simulink model "Braccio_CtrlSimMdl_2025b"  (R2025b)
settings: Solver=ode1  StartTime=0.0  StopTime=inf  FixedStep=dt  RelTol=1e-3  EnableMultiTasking=on
values from neighbouring files (symbols this model uses):
  dt = 0.01    [Braccio_ini.m]    (also in Braccio_kinematics.m)
  jnt1 = rigidBodyJoint('jnt1','revolute')    [Braccio_ini.m]    (also in Braccio_kinematics.m)
  jnt2 = rigidBodyJoint('jnt2','revolute')    [Braccio_ini.m]    (also in Braccio_kinematics.m)
  jnt3 = rigidBodyJoint('jnt3','revolute')    [Braccio_ini.m]    (also in Braccio_kinematics.m)
  jnt4 = rigidBodyJoint('jnt4','revolute')    [Braccio_ini.m]    (also in Braccio_kinematics.m)
  jnt5 = rigidBodyJoint('jnt5','revolute')    [Braccio_ini.m]    (also in Braccio_kinematics.m)
undefined symbols (not defined in the file or in its folder): DiscIntNeverNeededParam, efence1_coord, Gripper, Pause, Run
libraries: sim3dlib x22, Braccio_lib x12, simulink x12, robotmaniplib x1, stm32f4xxblockslib x1, robotcorelib x1, robotsim3dlib x1
(part 1 of 2)
settings Model: STM32="{\"DigitalPortRead\":[{\"ID\":\"MotorCtrl_Demo_STM32:8\"},{\"ID\":\"DemoSetup_H755ZIQ:8\"},{\"ID\":\"DemoSetup_H755ZIQ_M7:8\"},{\"ID\":\"Aktorik_H755ZIQ_M7:8\"},{\"ID\":\"IKS4A1_H755ZIQ_M7:8\"},{\"ID\":\"BlinkModel:8\"}],\"DigitalPortWrite\":[{\"ID\":\"MotorCtrl_Demo_STM32:9\"},{\"ID\":\"MotorCtrl_Demo_STM32:26\"},{\"ID\":\"MotorCtrl_Demo_STM32:27\"},{\"ID\":\"MotorCtrl_Demo_STM32:39\"},{\"ID\":\"MotorCtrl_Demo_STM32:489\"},{\"ID\":\"MotorCtrl_Demo_STM32:493\"},{\"ID\":\"MotorCtrl_Demo_STM32:582\"},{\"ID\":\"MotorCtrl_Demo_STM32:584\"},{\"ID\":\"MotorCtrl_Demo_STM32:585\"},{\"ID\":\"MotorCtrl_Demo_STM32:586\"},{\"ID\":\"DemoSetup_H755ZIQ:9\"},{\"ID\":\"DemoSetup_H755ZIQ_M7:9\"},{\"ID\":\"Aktorik_H755ZIQ_M7:9\"},{\"ID\":\"Aktorik_H755ZIQ_M7:886\"},{\"ID\":\"Aktorik_H755ZIQ_M7:887\"},{\"ID\":\"Aktorik_H755ZIQ_M7:929\"},{\"ID\":\"Aktorik_H755ZIQ_M7:930\"},{\"ID\":\"Aktorik_H755ZIQ_M7:1123\"},{\"ID\":\"Aktorik_H755ZIQ_M7:1128\"},{\"ID\":\"Aktorik_H755ZIQ_M7:1152\"},{\"ID\":\"Aktorik_H755ZIQ_M7:1176\"},{\"ID\":\"Aktorik_H755ZIQ_M7:1222\"},{\"ID\":\"Aktorik_H755ZIQ_M7:1224\"},{\"ID\":\"Aktorik_H755ZIQ_M7:1233\"},{\"ID\":\"IKS4A1_H755ZIQ_M7:9\"},{\"ID\":\"BlinkModel:9\"},{\"ID\":\"2666\"},{\"ID\":\"Braccio_CtrlSimMdl_2025b:2666\"}],\"PWMOutput\":[{\"ID\":\"MotorCtrl_Demo_STM32:23\"},{\"ID\":\"Aktorik_H755ZIQ_M7:885\"},{\"ID\":\"Aktorik_H755ZIQ_M7:988\"}],\"EncoderBlock\":[{\"ID\":\"MotorCtrl_Demo_STM32:41\"},{\"ID\":\"Aktorik_H755ZIQ_M7:1005\"}],\"AnalogInputForH7\":{\"ID\":\"Aktorik_H755ZIQ_M7:875\"},\"I2CControllerRead\":[{\"ID\":\"Aktorik_H755ZIQ_M7:1322\"},{\"ID\":\"Aktorik_H755ZIQ_M7:1414\"},{\"ID\":\"Aktorik_H755ZIQ_M7:1416\"},{\"ID\":\"Aktorik_H755ZIQ_M7:1435\"},{\"ID\":\"Aktorik_H755ZIQ_M7:1437\"},{\"ID\":\"Aktorik_H755ZIQ_M7:1438\"},{\"ID\":\"Aktorik_H755ZIQ_M7:1465\"},{\"ID\":\"Aktorik_H755ZIQ_M7:1466\"},{\"ID\":\"Aktorik_H755ZIQ_M7:1488\"},{\"ID\":\"Aktorik_H755ZIQ_M7:1489\"},{\"ID\":\"Aktorik_H755ZIQ_M7:1491\"},{\"ID\":\"Aktorik_H755ZIQ_M7:1492\"},{\"ID\":\"Aktorik_H755ZIQ_M7:1495\"},{\"ID\":\"Aktorik_H755ZIQ_M7:1496\"},{\"ID\":\"Aktorik_H755ZIQ_M7:1497\"},{\"ID\":\"Aktorik_H755ZIQ_M7:1498\"},{\"ID\":\"Aktorik_H755ZIQ_M7:1499\"},{\"ID\":\"Aktorik_H755ZIQ_M7:1500\"},{\"ID\":\"IKS4A1_H755ZIQ_M7:1435\"},{\"ID\":\"IKS4A1_H755ZIQ_M7:1437\"},{\"ID\":\"IKS4A1_H755ZIQ_M7:1438\"},{\"ID\":\"IKS4A1_H755ZIQ_M7:1414\"},{\"ID\":\"IKS4A1_H755ZIQ_M7:1416\"},{\"ID\":\"IKS4A1_H755ZIQ_M7:1495\"},{\"ID\":\"IKS4A1_H755ZIQ_M7:1496\"},{\"ID\":\"IKS4A1_H755ZIQ_M7:1497\"},{\"ID\":\"IKS4A1_H755ZIQ_M7:1498\"},{\"ID\":\"IKS4A1_H755ZIQ_M7:1499\"},{\"ID\":\"IKS4A1_H755ZIQ_M7:1500\"},{\"ID\":\"IKS4A1_H755ZIQ_M7:1465\"},{\"ID\":\"IKS4A1_H755ZIQ_M7:1466\"},{\"ID\":\"IKS4A1_H755ZIQ_M7:1488\"},{\"ID\":\"IKS4A1_H755ZIQ_M7:1489\"},{\"ID\":\"IKS4A1_H755ZIQ_M7:1491\"},{\"ID\":\"IKS4A1_H755ZIQ_M7:1492\"}],\"I2CControllerWrite\":[{\"ID\":\"Aktorik_H755ZIQ_M7:1375\"},{\"ID\":\"Aktorik_H755ZIQ_M7:1404\"},{\"ID\":\"Aktorik_H755ZIQ_M7:1452\"},{\"ID\":\"Aktorik_H755ZIQ_M7:1459\"},{\"ID\":\"Aktorik_H755ZIQ_M7:1511\"},{\"ID\":\"IKS4A1_H755ZIQ_M7:1404\"},{\"ID\":\"IKS4A1_H755ZIQ_M7:1375\"},{\"ID\":\"IKS4A1_H755ZIQ_M7:1452\"},{\"ID\":\"IKS4A1_H755ZIQ_M7:1511\"},{\"ID\":\"IKS4A1_H755ZIQ_M7:1459\"}]}"  ExtModeTrigDuration=10  Creator=bende  LastModifiedBy=natte
settings SolverCC: AutoInsertRateTranBlk=on
settings OptimizationCC: EnhancedBackFolding=on  PassReuseOutputArgsThreshold=0.0  MaxStackSize=256  OptimizeBlockOrder=speed  DifferentSizesBufferReuse=on  OptimizationCustomize=off
settings DebuggingCC: ParameterTunabilityLossMsg=error
settings HardwareCC: ProdBitPerLong=64.0  ProdHWDeviceType=Intel->x86-64 (Linux 64)  TargetBitPerPointer=64.0  TargetBitPerSizeT=64.0  TargetBitPerPtrDiffT=64.0  TargetLongLongMode=on  TargetIntDivRoundTo=Zero  TargetEndianess=LittleEndian  TargetWordSize=64.0  TargetHWDeviceType=MATLAB Host  ProdEqTarget=off
settings SFSimCC: MATLABDynamicMemAlloc=off
settings RTWCC: SystemTargetFile=rsim.tlc  TemplateMakefile=rsim_default_tmf  Toolchain=GNU Tools for ARM Embedded Processors  Description=Rapid Simulation Target
settings CodeAppCC: ForceParamTrailComments=on  MaxIdLength=95.0  OperatorAnnotations=on
settings STFCustomTargetCC: SystemTargetFile=rsim.tlc  TargetLangStandard=C99 (ISO)  ModelReferenceCompliant=off  ConcurrentExecutionCompliant=off  MATLABClassNameForMDSCustomization=Simulink.SoftwareTarget.TargetSpecificTriggerConfigurationBase
settings RSimTargetCC: ExtModeStaticAllocSize=1000000.0  ExtModeTransport=0.0  MultiwordLength=2048.0

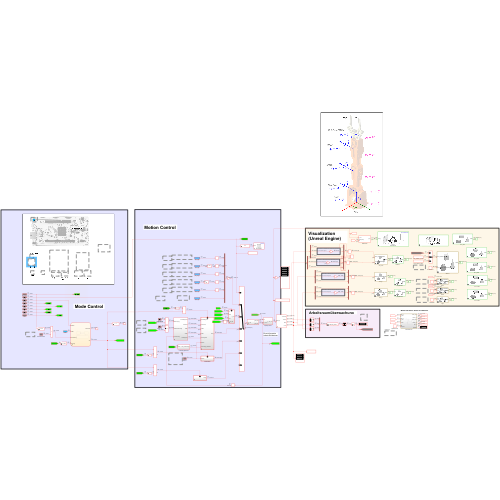
[thumbnail: Simulink's stored preview of the top-level diagram]
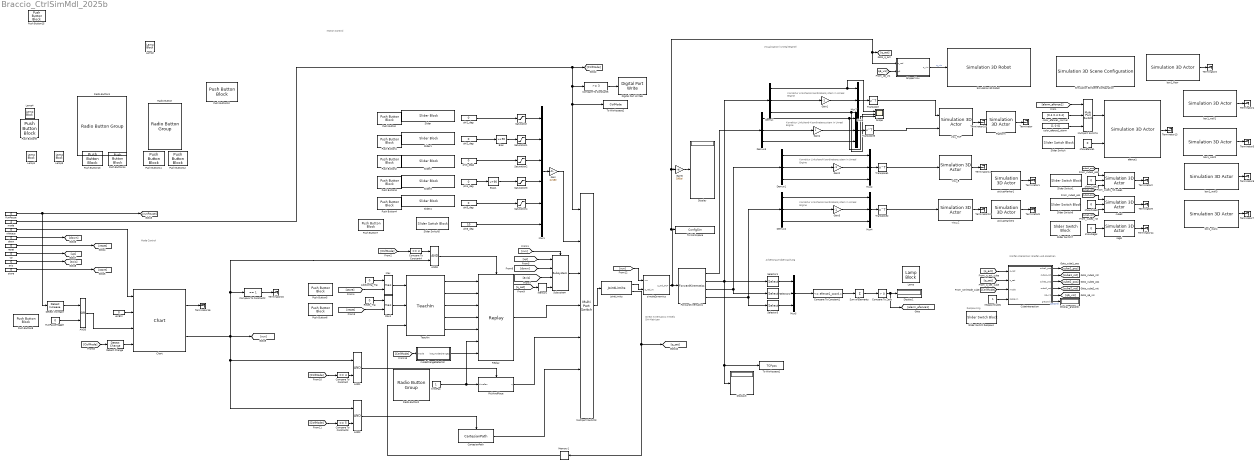
== system Braccio_CtrlSimMdl_2025b ==
  note: Korrektur Linkshand-Koordinatensystem
      | in Unreal Engine
  note: Arbeitsraumüberwachung
  note: Korrektur Linkshand-Koordinatensystem
      | in Unreal Engine
  note: Korrektur Linkshand-Koordinatensystem
      | in Unreal Engine
  note: Visualization
      | (Unreal Engine)
  note: Korrektur Linkshand-Koordinatensystem
      | in Unreal Engine
  note: Mode Control
  note: Motion Control
  note: Direct Kinematics
      | mittels DH-Matrizen
  note: Würfel-Interaktion: Greifen und Absetzen
  note: Respawning
  AND1 : Logic  AllPortsSameDT=off  OutDataTypeStr=boolean
  AND2 : Logic  AllPortsSameDT=off  OutDataTypeStr=boolean
  AND3 : Logic  AllPortsSameDT=off  OutDataTypeStr=boolean
  AND5 : Logic  Operator=OR  AllPortsSameDT=off  OutDataTypeStr=boolean
  AddConfig_Trg : Constant  Value=0  SampleTime=dt
  Bias : Bias  Bias=90  SaturateOnIntegerOverflow=off
  Bias1 : Bias  Bias=90  SaturateOnIntegerOverflow=off
  CartesianPath : Braccio_lib/CartesianPath  SystemSampleTime=-1  VariantActivationTime=update diagram  EmptyChoice=off  PassThrough=off  PassThroughVariantControl=(default)  EmptyChoiceVariantControl=(default)  AllowFlexibleInterface=on  Latency=0  AutoFrameSizeCalculation=off
  Chart : Braccio_lib/Chart  SystemSampleTime=-1  VariantActivationTime=update diagram  EmptyChoice=off  PassThrough=off  PassThroughVariantControl=(default)  EmptyChoiceVariantControl=(default)  AllowFlexibleInterface=on  Latency=0  AutoFrameSizeCalculation=off
  Compare To Constant : simulink/Logic and Bit Operations/Compare To Constant  relop===  const=4  OutDataTypeStr=boolean
  Compare To Constant1 : simulink/Logic and Bit Operations/Compare To Constant  relop=<=  const=efence1_coord.x  OutDataTypeStr=boolean
  Compare To Constant2 : simulink/Logic and Bit Operations/Compare To Constant  relop===  const=1  OutDataTypeStr=boolean
  Compare To Constant3 : simulink/Logic and Bit Operations/Compare To Constant  relop===  const=5  OutDataTypeStr=boolean
  Compare To Constant4 : simulink/Logic and Bit Operations/Compare To Constant  relop===  const=3  OutDataTypeStr=boolean
  Compare To Constant5 : simulink/Logic and Bit Operations/Compare To Constant  relop=>=  const=3  OutDataTypeStr=boolean
  Compare To Zero : simulink/Logic and Bit Operations/Compare To Zero  relop=>  OutDataTypeStr=boolean
  CubeInteraction : Subsystem
  Demux{,1..3} (4 alike) : Demux  Outputs=3
  Detect Change : simulink/Logic and Bit Operations/Detect Change  vinit=0  OutDataTypeStr=boolean
  Detect Increase : simulink/Logic and Bit Operations/Detect Increase  vinit=0.0  OutDataTypeStr=boolean
  Digital Port Write5 : stm32f4xxblockslib/Digital Port Write  PortName=GPIOD  PinNumber=7  ReadOperation=off  IOAsArray=off  EnableSimPort=off  hoistedMaskSrc=ECSoC/ECSimCodegen/Digital Port Write
      settings: LibrarySourceBlock=stm32h7xxblockslib/Digital Port Write
  Display : Display
  Display1 : Display
  Display3 : Display
  Display_graspIdx : Display
  ForwardKinematics : Braccio_lib/ForwardKinematics  SystemSampleTime=-1  VariantActivationTime=update diagram  EmptyChoice=off  PassThrough=off  PassThroughVariantControl=(default)  EmptyChoiceVariantControl=(default)  AllowFlexibleInterface=on  Latency=0  AutoFrameSizeCalculation=off
  Gain : Gain  Gain=pi/180
  Gain1 : Gain  Gain=-1
  Gain2 : Gain  Gain=-1
  Gain3 : Gain  Gain=-1
  Gain4 : Gain
  Gain5 : Gain  Gain=180/pi
  GripperVisu : MATLAB Function  TreatAsAtomicUnit=on
  JointLimits : Braccio_lib/JointLimits  SystemSampleTime=-1  VariantActivationTime=update diagram  EmptyChoice=off  PassThrough=off  PassThroughVariantControl=(default)  EmptyChoiceVariantControl=(default)  AllowFlexibleInterface=on  Latency=0  AutoFrameSizeCalculation=off
  Lamp{,1..4} (5 alike) : LampBlock  LabelPosition=Hide  DefaultColor=[192.0, 192.0, 192.0]
  Max : MinMax  Function=max  Inputs=2
  Max1 : MinMax  Function=max  Inputs=2
  Memory : Memory  InitialCondition=[0;90;0;90;0;20]*pi/180
  Memory1 : Memory  InheritSampleTime=on
  Multiport Switch1 : MultiPortSwitch  DataPortOrder=Zero-based contiguous  Inputs=2  zeroidx=on  SaturateOnIntegerOverflow=off  InputSameDT=off
  Multiport Switch3 : MultiPortSwitch  Inputs=6  SaturateOnIntegerOverflow=off  InputSameDT=off
  Mux1 : Mux  Inputs=6
  Mux{2..5,7} (5 alike) : Mux  Inputs=3
  PickAndPlace : Subsystem  AncestorBlock=Braccio_lib/PickAndPlace
  Platform : sim3dlib/Simulation 3D Actor  Priority=1  ActorName=actor1_platform  ParentName=Scene Origin  Operation=Create at setup  InitScriptText=|  SampleTime=-1  Translation=[0.1 0 -0.01]  Rotation=[0 0 0]  Scale=[1 1 1]  aMode=5  ActorTag=actor1_platform  ActorType=Sim3dActor  ID=C
      | % Reserved keywords:
      | % - Actor : handle to this actor object
      | % - World : handle to the world object
      | 
      | % Examples:
      | 
      | % Create a primitive geometry (optional)
      | createShape(Actor, 'box', [0.6,0.3,0.02]);
      | 
      | % Initialize values (optional)
      | Actor.Physics = false;
      | Actor.Color = [0.4 0.4 0.4];
      | %platform = collisionBox(0.6,0.3,0.02);
      | %platform.Pose = trvec2tform([-0.1 0 -.01]);
  Push Button : PushButtonBlock  ButtonText=Reset q1  OnValue=0  ButtonType=Latch  IconOnColor=[0.0, 0.39215686274509803, 0.0]  IconOffColor=[0.0, 1.0, 0.0]  OffValue=-2.550607
  Push Button1 : PushButtonBlock  ButtonText=Reset q2  OnValue=0  ButtonType=Latch  IconOnColor=[0.0, 0.39215686274509803, 0.0]  IconOffColor=[0.0, 1.0, 0.0]  OffValue=48.947368
  Push Button10 : PushButtonBlock  ButtonText=NOTAUS  Icon=Circle  IconOnColor=[1.0, 0.0, 0.0]  IconOffColor=[1.0, 0.0, 0.0]  IconColor=On  OffValue=0.000000
  Push Button{9,11..14} (5 alike) : PushButtonBlock  Icon=Circle  IconOnColor=[0.0, 0.39215686274509803, 0.0]  IconOffColor=[0.0, 1.0, 0.0]  OffValue=0.000000
  Push Button15 : PushButtonBlock  ButtonText=USR BTN  IconOnColor=[0.0, 0.39215686274509803, 0.0]  IconOffColor=[0.0, 1.0, 0.0]  OffValue=0.000000
  Push Button2 : PushButtonBlock  ButtonText=Reset q3  OnValue=0  ButtonType=Latch  IconOnColor=[0.0, 0.39215686274509803, 0.0]  IconOffColor=[0.0, 1.0, 0.0]  OffValue=-17.636995
  Push Button3 : PushButtonBlock  ButtonText=Reset q4  OnValue=0  ButtonType=Latch  IconOnColor=[0.0, 0.39215686274509803, 0.0]  IconOffColor=[0.0, 1.0, 0.0]  OffValue=-12.105263
  Push Button4 : PushButtonBlock  ButtonText=Reset q5  OnValue=0  ButtonType=Latch  IconOnColor=[0.0, 0.39215686274509803, 0.0]  IconOffColor=[0.0, 1.0, 0.0]  OffValue=-61.435656
  Push Button5 : PushButtonBlock  ButtonText=SAVE CONFIG  IconOnColor=[0.0, 0.39215686274509803, 0.0]  IconOffColor=[0.0, 1.0, 0.0]  OffValue=0.000000
  Push Button6 : PushButtonBlock  ButtonText=RESET  IconOnColor=[0.0, 0.39215686274509803, 0.0]  IconOffColor=[0.0, 1.0, 0.0]
  Push Button7 : PushButtonBlock  ButtonText=SAVE CONFIG  IconOnColor=[0.0, 0.39215686274509803, 0.0]  IconOffColor=[0.0, 1.0, 0.0]  OffValue=0.000000
  Push Button8 : PushButtonBlock  ButtonText=Run-Pause  IconOnColor=[0.0, 0.39215686274509803, 0.0]  IconOffColor=[0.0, 1.0, 0.0]  OffValue=0.000000
  Radio Button : RadioButtonGroup  LabelPosition=Hide  SelectedLabel=6 - Gripper  ButtonGroupName=Axis
  Radio Button1 : RadioButtonGroup  LabelPosition=Hide  SelectedLabel=Pick'n'Place  ButtonGroupName=Mode
  Radio Button2 : RadioButtonGroup  LabelPosition=Hide  SelectedLabel=Normal  ButtonGroupName=timeFac
  Replay : Braccio_lib/Replay  SystemSampleTime=-1  VariantActivationTime=update diagram  EmptyChoice=off  PassThrough=off  PassThroughVariantControl=(default)  EmptyChoiceVariantControl=(default)  AllowFlexibleInterface=on  Latency=0  AutoFrameSizeCalculation=off
  Reset_Trg : Constant  Value=0  SampleTime=dt
  RunPause : Constant  Value=0  SampleTime=dt
  RunPauseToggle : Constant  Value=0  SampleTime=dt
  Saturation : Saturate  UpperLimit=jnt1.PositionLimits(2)*180/pi  LowerLimit=jnt1.PositionLimits(1)*180/pi
  Saturation1 : Saturate  UpperLimit=jnt2.PositionLimits(2)*180/pi  LowerLimit=jnt2.PositionLimits(1)*180/pi
  Saturation2 : Saturate  UpperLimit=jnt3.PositionLimits(2)*180/pi  LowerLimit=jnt3.PositionLimits(1)*180/pi
  Saturation3 : Saturate  UpperLimit=jnt4.PositionLimits(2)*180/pi  LowerLimit=jnt4.PositionLimits(1)*180/pi
  Saturation4 : Saturate  UpperLimit=jnt5.PositionLimits(2)*180/pi  LowerLimit=jnt5.PositionLimits(1)*180/pi
  Scope : Scope  NumInputPorts=3
      settings: ActiveDisplayYMinimum=0.35929394467848708  ActiveDisplayYMaximum=0.36634551278284788  DataLoggingVariableName=ScopeData3
  Selector1 : Selector  InputPortWidth=3  IndexOptions=Index vector (dialog)  Indices=1  OutputSizes=1
  Selector2 : Selector  InputPortWidth=3  IndexOptions=Index vector (dialog)  Indices=1  OutputSizes=1
  Selector3 : Selector  InputPortWidth=3  IndexOptions=Index vector (dialog)  Indices=1  OutputSizes=1
  Simulation 3D Robot : robotsim3dlib/Simulation 3D Robot  actorInputType=RigidBodyTree Object  RigidBodyTree=braccioRobotVis  ActorName=braccioRobot  existActorChekBox=off  initialTrans=[0 0 0]  initialRot=[0 0 0]  initialConfig=braccioInitConfigVis  EndEffector=body5  eeOffsetInpChekBox=off  eeTargetTrans=[0 0 0]  eeTargetRot=[0 0 0]  enableRegionGraspChekBox=off  regionGraspInpChekBox=off  eeTargTransDiff=[0.2 0.2 0.2]  eeTargRotDiff=[0 0 0]  enableVisualVisualization=on  enableCollisionVisualization=on  collisionGeomColor=[0 1 0]  collisionGeomTransp=0.1  inpConfEnbVal=on  inpGraspEnbVal=off  inpTransEnbVal=off  outConfEnbVal=off  outGraspEnbVal=off  outTransEnbVal=off  SampleTime=-1  ActorType=SimulinkVehicle  ID=C  aMode=6  ActorTag=braccioRobot  Mesh=RigidBodyTree
  Simulation 3D Scene Configuration : sim3dlib/Simulation 3D Scene Configuration  Priority=0  ProjectFormat=Default Scenes  SceneDesc=Empty scene  ProjectName=C:\Program Files\MATLAB\R2025b\toolbox\shared\sim3d_projects\automotive_project_windows\UE\WindowsNoEditor\VehicleSimulation.exe  ScenePath=/Game/Maps/EmptyScene  EnableOpenDRIVE=off  vehTagList={'Actor_B';'Actor_C';'Actor_TCP';'Actor_efence1';'Custom';'Scene Origin';'Sim3dActor1';'View1';'View2';'View3';'View4';'actor1_platform';'actor2_pickupMarker';'actor_cube1';'actor_cube2';'actor_regal';'boxActor1';'boxActor2';'boxActor3';'boxActor4';'boxActor5';'braccioRobot'}  vehTag=View4  AttachedCameraRelativeTranslation=[0 0 0]  FreeCameraDefaultInitialTranslation=[-6, 0, 2]  AttachedCameraRelativeRotation=[0 0 0]  FreeCameraDefaultInitialRotation=[0, -15, 0]  ViewpointName=View4  FreeCameraInitialTranslation=[0.25 -0.4 0.4]  ViewpointTranslation=[0 0 0]  FreeCameraInitialRotation=[0 -35 110]  ViewpointRotation=[0 0 0]  OpVisEn=off  Ts=0.1  EnableWindow=on  EnableRemoteAccess=off  EnableWeather=on  SunAzimuth=90  SunAltitude=40.0  EnableGeospatialSun=off  Latitude=0  Longitude=0  Date=2023-01-01  Time=10:30:00  GeoTimeZone=-5.0  SunDaylightSaving=off  wind=0  clouds=0.0  EnableVolumetricClouds=off  CloudCoverage=0  CloudAltitude=6  fog=0  rain=0  RaindropsEffect=off  SnowDensity=0  EnableGeospatial=off  TilesetSource=Earth terrain  UseTrueOrigin=off  OriginHeight=200  OriginLatitude=40.744652  OriginLongitude=-73.988864  MapStyle=Aerial  AdditionalAssetIDs=[]  UseAdvancedSunSky=off  SolarTime=11  TimeZone=-5  Day=21  Month=9  Year=2022  UseDaylightSavingTime=on  DSTStartDay=10  DSTStartMonth=3  DSTEndDay=3  DSTEndMonth=11  DSTSwitchHour=2  sensorTag=MainCamera1  sensorId=1  sensorName=MainCamera1  mountLoc=Origin  offsetFlag=off  tmountOffset=[0, 0, 0]  rmountOffset=[0, 0, 0]  HorizontalResolution=1280  VerticalResolution=720  HorizontalFOV=60  mountPoint=[0 0 0]  mountOrientation=[0 0 0]  aMode=6  ID=1  GeoTrigger=Inactive  ViewNameList={'Custom', 'View1', 'View2', 'View3', 'View4'}  ViewTranslationList={'[0 -1 0]', '[-0.5 0 0.05]', '[0 -0.5 0.05]', '[0.15 0.5 0.25]', '[0.25 -0.4 0.4]'}  ViewRotationList={'[0 0 0]', '[0 0 0]', '[0 0 90]', '[0 -5 -90]', '[0 -35 110]'}
      settings: LibrarySourceBlock=robotsim3dlib/Simulation 3D Scene Configuration
  Slider{,1..4} (5 alike) : SliderBlock  ScaleMin=-90  ScaleMax=90
  Slider Switch{,1,5..7} (5 alike) : SliderSwitchBlock
  Slider Switch Respawn : SliderSwitchBlock
  Subsystem : Braccio_lib/Subsystem  SystemSampleTime=-1  VariantActivationTime=update diagram  EmptyChoice=off  PassThrough=off  PassThroughVariantControl=(default)  EmptyChoiceVariantControl=(default)  AllowFlexibleInterface=on  Latency=0  AutoFrameSizeCalculation=off
  Sum of Elements : Sum  Inputs=+
  TeachIn : Braccio_lib/TeachIn  SystemSampleTime=-1  VariantActivationTime=update diagram  EmptyChoice=off  PassThrough=off  PassThroughVariantControl=(default)  EmptyChoiceVariantControl=(default)  AllowFlexibleInterface=on  Latency=0  AutoFrameSizeCalculation=off
  Terminator{,1..16} (17 alike) : Terminator
  To Workspace : ToWorkspace  VariableName=ConfigSim  SaveFormat=Timeseries  SampleTime=-1
  To Workspace1 : ToWorkspace  VariableName=TCPpos  SaveFormat=Timeseries  SampleTime=-1
  To Workspace2 : ToWorkspace  VariableName=CtrlMode  SaveFormat=Timeseries  SampleTime=-1
  Transpose{,1..3} (4 alike) : Math  Operator=transpose
  axis : Constant  Value=6  SampleTime=dt
  box1_floor : sim3dlib/Simulation 3D Actor  Priority=1  ActorName=boxActor2  ParentName=Scene Origin  Operation=Create at setup  InitScriptText=|  SampleTime=-1  Translation=[0 -0.225 -.015]  Rotation=[0 0 0]  Scale=[1 1 1]  aMode=5  ActorTag=boxActor2  ActorType=Sim3dActor  ID=C
      | % Reserved keywords:
      | % - Actor : handle to this actor object
      | % - World : handle to the world object
      | 
      | % Examples:
      | 
      | % Create a primitive geometry (optional)
      | createShape(Actor, 'box', [0.1,0.15,0.005]);
      | 
      | % Initialize values (optional)
      | Actor.Physics = false;
      | Actor.Color = [0.4 0.4 0.4];
      | %platform = collisionBox(0.6,0.3,0.02);
      | %platform.Pose = trvec2tform([-0.1 0 -.01]);
  box1_wall1 : sim3dlib/Simulation 3D Actor  Priority=1  ActorName=boxActor3  ParentName=Scene Origin  Operation=Create at setup  InitScriptText=|  SampleTime=-1  Translation=[0 -0.15 .05-0.02]  Rotation=[0 0 0]  Scale=[1 1 1]  aMode=5  ActorTag=boxActor3  ActorType=Sim3dActor  ID=C
      | % Reserved keywords:
      | % - Actor : handle to this actor object
      | % - World : handle to the world object
      | 
      | % Examples:
      | 
      | % Create a primitive geometry (optional)
      | createShape(Actor, 'box', [0.1,0.005,0.1]);
      | 
      | % Initialize values (optional)
      | Actor.Physics = false;
      | Actor.Color = [0.4 0.4 0.4];
      | %platform = collisionBox(0.6,0.3,0.02);
      | %platform.Pose = trvec2tform([-0.1 0 -.01]);
  box1_wall2 : sim3dlib/Simulation 3D Actor  Priority=1  ActorName=boxActor4  ParentName=Scene Origin  Operation=Create at setup  InitScriptText=|  SampleTime=-1  Translation=[0 -0.3 .05-0.02]  Rotation=[0 0 0]  Scale=[1 1 1]  aMode=5  ActorTag=boxActor4  ActorType=Sim3dActor  ID=C
      | % Reserved keywords:
      | % - Actor : handle to this actor object
      | % - World : handle to the world object
      | 
      | % Examples:
      | 
      | % Create a primitive geometry (optional)
      | createShape(Actor, 'box', [0.1,0.005,0.1]);
      | 
      | % Initialize values (optional)
      | Actor.Physics = false;
      | Actor.Color = [0.4 0.4 0.4];
      | %platform = collisionBox(0.6,0.3,0.02);
      | %platform.Pose = trvec2tform([-0.1 0 -.01]);
  box1_wall3 : sim3dlib/Simulation 3D Actor  Priority=1  ActorName=boxActor5  ParentName=Scene Origin  Operation=Create at setup  InitScriptText=|  SampleTime=-1  Translation=[0.05 -0.225 0.05-0.02]  Rotation=[0 0 0]  Scale=[1 1 1]  aMode=5  ActorTag=boxActor5  ActorType=Sim3dActor  ID=C
      | % Reserved keywords:
      | % - Actor : handle to this actor object
      | % - World : handle to the world object
      | 
      | % Examples:
      | 
      | % Create a primitive geometry (optional)
      | createShape(Actor, 'box', [0.005,0.15,0.1]);
      | 
      | % Initialize values (optional)
      | Actor.Physics = false;
      | Actor.Color = [0.4 0.4 0.4];
      | %platform = collisionBox(0.6,0.3,0.02);
      | %platform.Pose = trvec2tform([-0.1 0 -.01]);
  box1_wall4 : sim3dlib/Simulation 3D Actor  Priority=1  ActorName=boxActor1  ParentName=Scene Origin  Operation=Create at setup  InitScriptText=|  SampleTime=-1  Translation=[-0.05 -0.225 0.05-0.02]  Rotation=[0 0 0]  Scale=[1 1 1]  aMode=5  ActorTag=boxActor1  ActorType=Sim3dActor  ID=C
      | % Reserved keywords:
      | % - Actor : handle to this actor object
      | % - World : handle to the world object
      | 
      | % Examples:
      | 
      | % Create a primitive geometry (optional)
      | createShape(Actor, 'box', [0.005,0.15,0.1]);
      | 
      | % Initialize values (optional)
      | Actor.Physics = false;
      | Actor.Color = [0.4 0.4 0.4];
      | %platform = collisionBox(0.6,0.3,0.02);
      | %platform.Pose = trvec2tform([-0.1 0 -.01]);
  color_efence1_alarm : Constant  Value=[1 0 0]  SampleTime=dt
  color_efence1_normal : Constant  Value=[0.4 0.4 0.4]  SampleTime=dt
  cube1 : sim3dlib/Simulation 3D Actor  Priority=1  ActorName=actor_cube1  ParentName=Scene Origin  Operation=Create at setup  InitScriptText=|  SampleTime=-1  Translation=[0.25 0 0.025/2+0.005]  Rotation=[0 0 0]  Scale=[1 1 1]  InputsText=|  aMode=5  ActorTag=actor_cube1  ActorType=Sim3dActor  ID=C
      InitScriptText=|
      | % Reserved keywords:
      | % - Actor : handle to this actor object
      | % - World : handle to the world object
      | 
      | % Examples:
      | 
      | % Create a primitive geometry (optional)
      | createShape(Actor, 'box', [0.025,0.025,0.025]);
      | 
      | % Initialize values (optional)
      | Actor.Physics = false;
      | Actor.Color = [0 0 1];
      | %platform = collisionBox(0.6,0.3,0.02);
      | %platform.Pose = trvec2tform([-0.1 0 -.01]);
      InputsText=|
      | actor_cube1.Translation
      | actor_cube1.Transparency
      | actor_cube1.Rotation
  cube2 : sim3dlib/Simulation 3D Actor  Priority=1  ActorName=actor_cube2  ParentName=Scene Origin  Operation=Create at setup  InitScriptText=|  SampleTime=-1  Translation=[0.35 0 0.025/2+0.005]  Rotation=[0 0 0]  Scale=[1 1 1]  InputsText=|  aMode=5  ActorTag=actor_cube2  ActorType=Sim3dActor  ID=C
      InitScriptText=|
      | % Reserved keywords:
      | % - Actor : handle to this actor object
      | % - World : handle to the world object
      | 
      | % Examples:
      | 
      | % Create a primitive geometry (optional)
      | createShape(Actor, 'box', [0.025,0.025,0.025]);
      | 
      | % Initialize values (optional)
      | Actor.Physics = false;
      | Actor.Color = [0 1 0];
      | %platform = collisionBox(0.6,0.3,0.02);
      | %platform.Pose = trvec2tform([-0.1 0 -.01]);
      InputsText=|
      | actor_cube2.Translation
      | actor_cube2.Transparency
      | actor_cube2.Rotation
  down : Constant  Value=0  SampleTime=dt
  efence1 : sim3dlib/Simulation 3D Actor  Priority=1  ActorName=Actor_efence1  ParentName=Scene Origin  Operation=Create at setup  InitScriptText=|  SampleTime=-1  Translation=[efence1_coord.x 0 0.15]  Rotation=[0 0 0]  Scale=[1 1 1]  InputsText="Actor_efence1.Color        Actor_efence1.Transparency"  aMode=5  ActorTag=Actor_efence1  ActorType=Sim3dActor  ID=C
      | % Reserved keywords:
      | % - Actor : handle to this actor object
      | % - World : handle to the world object
      | 
      | % Examples:
      | 
      | % Create a primitive geometry (optional)
      | createShape(Actor, 'box', [0.002,0.3,0.3]);
      | 
      | % Initialize values (optional)
      | Actor.Physics = false;
      | Actor.Color = [0.4 0.4 0.4];
      | Actor.Transparency = 0.4;
      | %platform = collisionBox(0.6,0.3,0.02);
      | %platform.Pose = trvec2tform([-0.1 0 -.01]);
  mode : Constant  Value=4  SampleTime=dt
  modeChangeDetector : Subsystem
  phi1_deg : Constant  Value=0  SampleTime=dt
  phi2_deg : Constant  Value=0  VectorParams1D=off  SampleTime=dt
  phi3_deg1 : Constant  Value=0  SampleTime=dt
  phi4_deg : Constant  Value=0  SampleTime=dt
  phi5_deg : Constant  Value=0  SampleTime=dt
  phi6_deg : Constant  Value=10  SampleTime=dt
  pickupMarker1 : sim3dlib/Simulation 3D Actor  Priority=1  ActorName=actor2_pickupMarker  ParentName=Scene Origin  Operation=Create at setup  InitScriptText=|  SampleTime=-1  Translation=[0.25 0 -.005]  Rotation=[0 0 0]  Scale=[1 1 1]  aMode=5  ActorTag=actor2_pickupMarker  ActorType=Sim3dActor  ID=C
      | % Reserved keywords:
      | % - Actor : handle to this actor object
      | % - World : handle to the world object
      | 
      | % Examples:
      | 
      | % Create a primitive geometry (optional)
      | createShape(Actor, 'box', [0.025,0.025,0.012]);
      | 
      | % Initialize values (optional)
      | Actor.Physics = false;
      | Actor.Color = [0.3 0.3 0.3];
      | %platform = collisionBox(0.6,0.3,0.02);
      | %platform.Pose = trvec2tform([-0.1 0 -.01]);
  pickupMarker2 : sim3dlib/Simulation 3D Actor  Priority=1  ActorName=Sim3dActor1  ParentName=Scene Origin  Operation=Create at setup  InitScriptText=|  SampleTime=-1  Translation=[0.35 0 -.005]  Rotation=[0 0 0]  Scale=[1 1 1]  aMode=5  ActorTag=Sim3dActor1  ActorType=Sim3dActor  ID=1
      | % Reserved keywords:
      | % - Actor : handle to this actor object
      | % - World : handle to the world object
      | 
      | % Examples:
      | 
      | % Create a primitive geometry (optional)
      | createShape(Actor, 'box', [0.025,0.025,0.012]);
      | 
      | % Initialize values (optional)
      | Actor.Physics = false;
      | Actor.Color = [0.3 0.3 0.3];
      | %platform = collisionBox(0.6,0.3,0.02);
      | %platform.Pose = trvec2tform([-0.1 0 -.01]);
  regal : sim3dlib/Simulation 3D Actor  Priority=1  ActorName=actor_regal  ParentName=Scene Origin  Operation=Create at setup  InitScriptText=|  SampleTime=-1  Translation=[0.4 0 0.05]  Rotation=[0 0 0]  Scale=[1 1 1]  InputsText=actor_regal.Transparency  aMode=5  ActorTag=actor_regal  ActorType=Sim3dActor  ID=C
      | % Reserved keywords:
      | % - Actor : handle to this actor object
      | % - World : handle to the world object
      | 
      | % Examples:
      | 
      | % Create a primitive geometry (optional)
      | createShape(Actor, 'box', [0.04,0.06,0.1]);
      | 
      | % Initialize values (optional)
      | Actor.Physics = false;
      | Actor.Color = [0.3 0.3 0.3];
      | %platform = collisionBox(0.6,0.3,0.02);
      | %platform.Pose = trvec2tform([-0.1 0 -.01]);
  reset : Constant  Value=0  SampleTime=dt
  respawnCubes : Constant  OutDataTypeStr=double  SampleTime=dt
  showCube1 : Constant  Value=0  SampleTime=dt
  showCube2 : Constant  Value=0  SampleTime=dt
  showEfence1 : Constant  Value=0  SampleTime=dt
  showRegal : Constant  Value=0  SampleTime=dt
  simpleDynamics : Subsystem
  store : Constant  Value=0  SampleTime=dt
  timeFac : Constant  SampleTime=dt
  up : Constant  Value=0  SampleTime=dt
  usrBtn : Constant  Value=0  SampleTime=dt
  visu_B : sim3dlib/Simulation 3D Actor  Priority=1  ActorName=Actor_B  ParentName=Scene Origin  Operation=Create at setup  InitScriptText=|  SampleTime=-1  Translation=box_trans  Rotation=[0 0 0]  Scale=[1 1 1]  InputsText=Actor_B.Translation  aMode=5  ActorTag=Actor_B  ActorType=Sim3dActor  ID=C
      | % Reserved keywords:
      | % - Actor : handle to this actor object
      | % - World : handle to the world object
      | 
      | % Examples:
      | 
      | % Create a primitive geometry (optional)
      | createShape(Actor, 'sphere', [0.01,0.01,0.01]);
      | 
      | % Initialize values (optional)
      | Actor.Physics = false;
      | Actor.Color = [1 0 0];
      | %platform = collisionBox(0.6,0.3,0.02);
      | %platform.Pose = trvec2tform([-0.1 0 -.01]);
  visu_C : sim3dlib/Simulation 3D Actor  Priority=1  ActorName=Actor_C  ParentName=Scene Origin  Operation=Create at setup  InitScriptText=|  SampleTime=-1  Translation=box_trans  Rotation=[0 0 0]  Scale=[1 1 1]  InputsText=Actor_C.Translation  aMode=5  ActorTag=Actor_C  ActorType=Sim3dActor  ID=C
      | % Reserved keywords:
      | % - Actor : handle to this actor object
      | % - World : handle to the world object
      | 
      | % Examples:
      | 
      | % Create a primitive geometry (optional)
      | createShape(Actor, 'sphere', [0.01,0.01,0.01]);
      | 
      | % Initialize values (optional)
      | Actor.Physics = false;
      | Actor.Color = [1 0 0];
      | %platform = collisionBox(0.6,0.3,0.02);
      | %platform.Pose = trvec2tform([-0.1 0 -.01]);
  visu_TCP : sim3dlib/Simulation 3D Actor  Priority=1  ActorName=Actor_TCP  ParentName=Scene Origin  Operation=Create at setup  InitScriptText=|  SampleTime=-1  Translation=box_trans  Rotation=[0 0 0]  Scale=[1 1 1]  InputsText=Actor_TCP.Translation Actor_TCP.Rotation  aMode=5  ActorTag=Actor_TCP  ActorType=Sim3dActor  ID=C
      | % Reserved keywords:
      | % - Actor : handle to this actor object
      | % - World : handle to the world object
      | 
      | % Examples:
      | 
      | % Create a primitive geometry (optional)
      | createShape(Actor, 'sphere', [0.01,0.01,0.01]);
      | 
      | % Initialize values (optional)
      | Actor.Physics = false;
      | Actor.Color = [1 0 0];
      | %platform = collisionBox(0.6,0.3,0.02);
      | %platform.Pose = trvec2tform([-0.1 0 -.01]);
  xNotaus : Constant  Value=0  SampleTime=dt
  wires:
  Platform/1 -> Terminator/1
  pickupMarker1/1 -> Terminator1/1
  cube1/1 -> Terminator2/1
  box1_floor/1 -> Terminator3/1
  box1_wall1/1 -> Terminator4/1
  box1_wall2/1 -> Terminator5/1
  box1_wall3/1 -> Terminator6/1
  box1_wall4/1 -> Terminator7/1
  Mux3/1 -> Transpose/1
  Demux/3 -> Scope/2, Mux3/3
  Demux/2 -> Gain1/1
  Demux/1 -> Scope/1, Mux3/1
  Gain1/1 -> Mux3/2
  ForwardKinematics/2 -> Demux/1, Selector1/1, Display3/1, To Workspace1/1
  visu_TCP/1 -> Terminator10/1
  visu_B/1 -> Terminator11/1
  ForwardKinematics/3 -> Demux1/1, Selector2/1
  Gain2/1 -> Mux2/2
  Demux1/1 -> Mux2/1
  Demux1/2 -> Gain2/1
  Demux1/3 -> Mux2/3
  Mux2/1 -> Transpose1/1
  Mux4/1 -> Transpose2/1
  Demux2/3 -> Mux4/3
  Demux2/2 -> Gain3/1
  Gain3/1 -> Mux4/2
  ForwardKinematics/4 -> Demux2/1, Selector3/1
  visu_C/1 -> Terminator12/1
  Demux2/1 -> Mux4/1
  efence1/1 -> Terminator13/1
  Selector1/1 -> Mux5/1
  Selector2/1 -> Mux5/2
  Selector3/1 -> Mux5/3
  Mux5/1 -> Compare To Constant1/1
  Compare To Constant1/1 -> Sum of Elements/1
  Sum of Elements/1 -> Compare To Zero/1
  Compare To Zero/1 -> [alarm_efence1], Display1/1
  Multiport Switch1/1 -> efence1/1
  [alarm_efence1] -> Multiport Switch1/1
  color_efence1_normal/1 -> Multiport Switch1/2
  color_efence1_alarm/1 -> Multiport Switch1/3
  showEfence1/1 -> efence1/2
  ForwardKinematics/1 -> Demux3/1
  Gain4/1 -> Mux7/2
  Demux3/1 -> Scope/3, Mux7/1
  Demux3/2 -> Gain4/1
  Demux3/3 -> Mux7/3
  Mux7/1 -> Transpose3/1
  Transpose/1 -> visu_TCP/1
  Transpose3/1 -> visu_TCP/2
  pickupMarker2/1 -> Terminator8/1
  cube2/1 -> Terminator9/1
  regal/1 -> Terminator14/1
  showRegal/1 -> regal/1
  CartesianPath/1 -> Multiport Switch3/6
  AND5/1 -> Chart/3
  Chart/2 -> AND2/1, AND1/1, [run], AND3/2, Compare To Constant2/1
  usrBtn/1 -> Chart/2
  Chart/1 -> Terminator16/1
  Detect Change/1 -> Chart/4
  [CtrlMode] -> Compare To Constant3/1
  xNotaus/1 -> Chart/1
  [axis] -> Subsystem/3
  Memory/1 -> Subsystem/4
  [run] -> Subsystem/Enable
  [up] -> Subsystem/1
  [down] -> Subsystem/2
  Subsystem/1 -> Multiport Switch3/3
  [CtrlMode] -> Compare To Constant/1
  Replay/1 -> Multiport Switch3/4
  Bias/1 -> Saturation1/1
  phi4_deg/1 -> Bias1/1
  Saturation3/1 -> Mux1/4
  TeachIn/4 -> Replay/4
  phi1_deg/1 -> Saturation/1
  down/1 -> [down]
  AddConfig_Trg/1 -> Max/1
  phi6_deg/1 -> Mux1/6
  JointLimits/1 -> simpleDynamics/2(q_rad_IN)
  Saturation/1 -> Mux1/1
  phi5_deg/1 -> Saturation4/1
  Compare To Constant/1 -> AND1/2
  phi3_deg1/1 -> Saturation2/1
  AND3/1 -> Replay/Enable
  TeachIn/5 -> Replay/5
  Saturation2/1 -> Mux1/3
  AND1/1 -> PickAndPlace/Enable
  Compare To Constant3/1 -> AND2/2
  [CtrlMode] -> Compare To Constant4/1
  Saturation1/1 -> Mux1/2
  Compare To Constant2/1 -> Terminator15/1
  mode/1 -> Multiport Switch3/1, To Workspace2/1, Compare To Constant5/1, [CtrlMode]
  Multiport Switch3/1 -> JointLimits/1
  axis/1 -> [axis]
  Mux1/1 -> Gain/1
  [store] -> Max/2
  [q_set] -> Memory/1
  Gain5/1 -> Display/1
  TeachIn/1 -> Replay/1
  RunPauseToggle/1 -> AND5/2
  Reset_Trg/1 -> Max1/1
  phi2_deg/1 -> Bias/1
  up/1 -> [up]
  Max/1 -> TeachIn/1
  [CtrlMode] -> Detect Change/1
  Memory1/1 -> TeachIn/3
  Compare To Constant5/1 -> Digital Port Write5/1
  Compare To Constant4/1 -> AND3/1
  Max1/1 -> TeachIn/2
  RunPause/1 -> [runPause], Detect Increase/1
  JointLimits/2 -> [q_set], Memory1/1
  [reset] -> Max1/2
  TeachIn/2 -> Replay/2
  Gain/1 -> Multiport Switch3/2
  Detect Increase/1 -> AND5/1
  Saturation4/1 -> Mux1/5
  TeachIn/3 -> Replay/3
  Bias1/1 -> Saturation3/1
  PickAndPlace/1(q) -> Multiport Switch3/5
  AND2/1 -> CartesianPath/Enable
  reset/1 -> [reset]
  store/1 -> [store]
  simpleDynamics/1(q_rad_OUT) -> ForwardKinematics/1, To Workspace/1, Gain5/1, GripperVisu/1(q_rad), [q_act]
  [run] -> simpleDynamics/1(run)
  Transpose1/1 -> visu_B/1
  Transpose2/1 -> visu_C/1
  timeFac/1 -> Replay/6, PickAndPlace/1(timeFac)
  [CtrlMode] -> modeChangeDetector/1(mode)
  modeChangeDetector/1(last_modeChanges) -> Replay/7
  [q6_vis] -> GripperVisu/2(q6)
  GripperVisu/1(q_vis) -> Simulation 3D Robot/1  "q_vis"
  [q_act] -> CubeInteraction/1(q_rad)
  [q_set] -> CubeInteraction/2(q_set)
  [CtrlMode] -> CubeInteraction/3(mode)
  CubeInteraction/1(cube1_pos) -> [cube1_pos]
  CubeInteraction/2(cube1_rot) -> [cube1_rot]
  CubeInteraction/3(cube2_pos) -> [cube2_pos]
  CubeInteraction/4(cube2_rot) -> [cube2_rot]
  CubeInteraction/5(q6_vis) -> [q6_vis]
  CubeInteraction/6(graspIdx) -> Display_graspIdx/1  "graspIdx"
  showCube1/1 -> cube1/2
  showCube2/1 -> cube2/2
  [cube1_pos] -> cube1/1
  [cube1_rot] -> cube1/3
  [cube2_pos] -> cube2/1
  [cube2_rot] -> cube2/3
  respawnCubes/1 -> CubeInteraction/4(respawn)

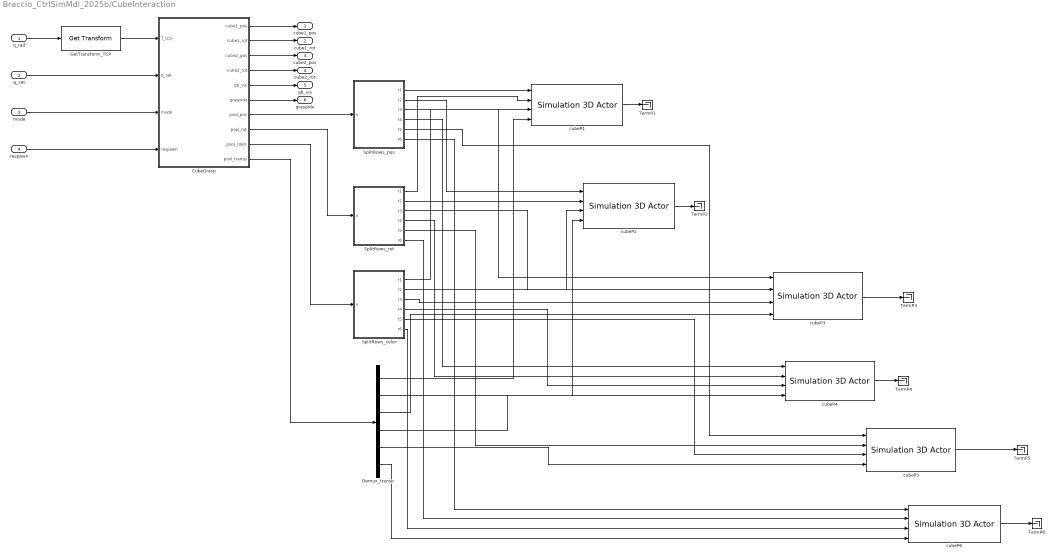
== system Braccio_CtrlSimMdl_2025b/CubeInteraction ==
  q_rad : Inport
  q_set : Inport  Port=2
  mode : Inport  Port=3
  respawn : Inport  Port=4
  CubeGrasp : MATLAB Function  TreatAsAtomicUnit=on
  Demux_transp : Demux  Outputs=6
  GetTransform_TCP : robotmaniplib/Get Transform  RigidBodyTree=braccioRobot  SourceBody=tcp  TargetBody=base  SimulateUsing=Interpreted execution
  SplitRows_color : MATLAB Function  TreatAsAtomicUnit=on
  SplitRows_pos : MATLAB Function  TreatAsAtomicUnit=on
  SplitRows_rot : MATLAB Function  TreatAsAtomicUnit=on
  TermP{1..6} (6 alike) : Terminator
  cubeP1 : sim3dlib/Simulation 3D Actor  Priority=1  ActorName=actor_cubeP1  ParentName=Scene Origin  Operation=Create at setup  InitScriptText=|  SampleTime=-1  Translation=[0 0 -1]  Rotation=[0 0 0]  Scale=[1 1 1]  InputsText=|  aMode=5  ActorTag=actor_cubeP1  ActorType=Sim3dActor  ID=C
      InitScriptText=|
      | % Reserved keywords:
      | % - Actor : handle to this actor object
      | % - World : handle to the world object
      | 
      | % Examples:
      | 
      | % Create a primitive geometry (optional)
      | createShape(Actor, 'box', [0.025,0.025,0.025]);
      | 
      | % Initialize values (optional)
      | Actor.Physics = false;
      | Actor.Color = [0 0 1];
      | %platform = collisionBox(0.6,0.3,0.02);
      | %platform.Pose = trvec2tform([-0.1 0 -.01]);
      InputsText=|
      | actor_cubeP1.Translation
      | actor_cubeP1.Rotation
      | actor_cubeP1.Color
      | actor_cubeP1.Transparency
  cubeP2 : sim3dlib/Simulation 3D Actor  Priority=1  ActorName=actor_cubeP2  ParentName=Scene Origin  Operation=Create at setup  InitScriptText=|  SampleTime=-1  Translation=[0 0 -1]  Rotation=[0 0 0]  Scale=[1 1 1]  InputsText=|  aMode=5  ActorTag=actor_cubeP2  ActorType=Sim3dActor  ID=C
      InitScriptText=|
      | % Reserved keywords:
      | % - Actor : handle to this actor object
      | % - World : handle to the world object
      | 
      | % Examples:
      | 
      | % Create a primitive geometry (optional)
      | createShape(Actor, 'box', [0.025,0.025,0.025]);
      | 
      | % Initialize values (optional)
      | Actor.Physics = false;
      | Actor.Color = [0 0 1];
      | %platform = collisionBox(0.6,0.3,0.02);
      | %platform.Pose = trvec2tform([-0.1 0 -.01]);
      InputsText=|
      | actor_cubeP2.Translation
      | actor_cubeP2.Rotation
      | actor_cubeP2.Color
      | actor_cubeP2.Transparency
  cubeP3 : sim3dlib/Simulation 3D Actor  Priority=1  ActorName=actor_cubeP3  ParentName=Scene Origin  Operation=Create at setup  InitScriptText=|  SampleTime=-1  Translation=[0 0 -1]  Rotation=[0 0 0]  Scale=[1 1 1]  InputsText=|  aMode=5  ActorTag=actor_cubeP3  ActorType=Sim3dActor  ID=C
      InitScriptText=|
      | % Reserved keywords:
      | % - Actor : handle to this actor object
      | % - World : handle to the world object
      | 
      | % Examples:
      | 
      | % Create a primitive geometry (optional)
      | createShape(Actor, 'box', [0.025,0.025,0.025]);
      | 
      | % Initialize values (optional)
      | Actor.Physics = false;
      | Actor.Color = [0 0 1];
      | %platform = collisionBox(0.6,0.3,0.02);
      | %platform.Pose = trvec2tform([-0.1 0 -.01]);
      InputsText=|
      | actor_cubeP3.Translation
      | actor_cubeP3.Rotation
      | actor_cubeP3.Color
      | actor_cubeP3.Transparency
  cubeP4 : sim3dlib/Simulation 3D Actor  Priority=1  ActorName=actor_cubeP4  ParentName=Scene Origin  Operation=Create at setup  InitScriptText=|  SampleTime=-1  Translation=[0 0 -1]  Rotation=[0 0 0]  Scale=[1 1 1]  InputsText=|  aMode=5  ActorTag=actor_cubeP4  ActorType=Sim3dActor  ID=C
      InitScriptText=|
      | % Reserved keywords:
      | % - Actor : handle to this actor object
      | % - World : handle to the world object
      | 
      | % Examples:
      | 
      | % Create a primitive geometry (optional)
      | createShape(Actor, 'box', [0.025,0.025,0.025]);
      | 
      | % Initialize values (optional)
      | Actor.Physics = false;
      | Actor.Color = [0 0 1];
      | %platform = collisionBox(0.6,0.3,0.02);
      | %platform.Pose = trvec2tform([-0.1 0 -.01]);
      InputsText=|
      | actor_cubeP4.Translation
      | actor_cubeP4.Rotation
      | actor_cubeP4.Color
      | actor_cubeP4.Transparency
  cubeP5 : sim3dlib/Simulation 3D Actor  Priority=1  ActorName=actor_cubeP5  ParentName=Scene Origin  Operation=Create at setup  InitScriptText=|  SampleTime=-1  Translation=[0 0 -1]  Rotation=[0 0 0]  Scale=[1 1 1]  InputsText=|  aMode=5  ActorTag=actor_cubeP5  ActorType=Sim3dActor  ID=C
      InitScriptText=|
      | % Reserved keywords:
      | % - Actor : handle to this actor object
      | % - World : handle to the world object
      | 
      | % Examples:
      | 
      | % Create a primitive geometry (optional)
      | createShape(Actor, 'box', [0.025,0.025,0.025]);
      | 
      | % Initialize values (optional)
      | Actor.Physics = false;
      | Actor.Color = [0 0 1];
      | %platform = collisionBox(0.6,0.3,0.02);
      | %platform.Pose = trvec2tform([-0.1 0 -.01]);
      InputsText=|
      | actor_cubeP5.Translation
      | actor_cubeP5.Rotation
      | actor_cubeP5.Color
      | actor_cubeP5.Transparency
  cubeP6 : sim3dlib/Simulation 3D Actor  Priority=1  ActorName=actor_cubeP6  ParentName=Scene Origin  Operation=Create at setup  InitScriptText=|  SampleTime=-1  Translation=[0 0 -1]  Rotation=[0 0 0]  Scale=[1 1 1]  InputsText=|  aMode=5  ActorTag=actor_cubeP6  ActorType=Sim3dActor  ID=C
      InitScriptText=|
      | % Reserved keywords:
      | % - Actor : handle to this actor object
      | % - World : handle to the world object
      | 
      | % Examples:
      | 
      | % Create a primitive geometry (optional)
      | createShape(Actor, 'box', [0.025,0.025,0.025]);
      | 
      | % Initialize values (optional)
      | Actor.Physics = false;
      | Actor.Color = [0 0 1];
      | %platform = collisionBox(0.6,0.3,0.02);
      | %platform.Pose = trvec2tform([-0.1 0 -.01]);
      InputsText=|
      | actor_cubeP6.Translation
      | actor_cubeP6.Rotation
      | actor_cubeP6.Color
      | actor_cubeP6.Transparency
  cube1_pos : Outport
  cube1_rot : Outport  Port=2
  cube2_pos : Outport  Port=3
  cube2_rot : Outport  Port=4
  q6_vis : Outport  Port=5
  graspIdx : Outport  Port=6
  wires:
  q_rad/1 -> GetTransform_TCP/1
  GetTransform_TCP/1 -> CubeGrasp/1(T_tcp)
  q_set/1 -> CubeGrasp/2(q_set)
  mode/1 -> CubeGrasp/3(mode)
  respawn/1 -> CubeGrasp/4(respawn)
  CubeGrasp/1(cube1_pos) -> cube1_pos/1
  CubeGrasp/2(cube1_rot) -> cube1_rot/1
  CubeGrasp/3(cube2_pos) -> cube2_pos/1
  CubeGrasp/4(cube2_rot) -> cube2_rot/1
  CubeGrasp/5(q6_vis) -> q6_vis/1
  CubeGrasp/6(graspIdx) -> graspIdx/1
  CubeGrasp/10(pool_transp) -> Demux_transp/1
  Demux_transp/1 -> cubeP1/4
  cubeP1/1 -> TermP1/1
  Demux_transp/2 -> cubeP2/4
  cubeP2/1 -> TermP2/1
  Demux_transp/3 -> cubeP3/4
  cubeP3/1 -> TermP3/1
  Demux_transp/4 -> cubeP4/4
  cubeP4/1 -> TermP4/1
  Demux_transp/5 -> cubeP5/4
  cubeP5/1 -> TermP5/1
  Demux_transp/6 -> cubeP6/4
  cubeP6/1 -> TermP6/1
  CubeGrasp/7(pool_pos) -> SplitRows_pos/1(v)
  SplitRows_pos/1(r1) -> cubeP1/1
  SplitRows_pos/2(r2) -> cubeP2/1
  SplitRows_pos/3(r3) -> cubeP3/1
  SplitRows_pos/4(r4) -> cubeP4/1
  SplitRows_pos/5(r5) -> cubeP5/1
  SplitRows_pos/6(r6) -> cubeP6/1
  CubeGrasp/8(pool_rot) -> SplitRows_rot/1(v)
  SplitRows_rot/1(r1) -> cubeP1/2
  SplitRows_rot/2(r2) -> cubeP2/2
  SplitRows_rot/3(r3) -> cubeP3/2
  SplitRows_rot/4(r4) -> cubeP4/2
  SplitRows_rot/5(r5) -> cubeP5/2
  SplitRows_rot/6(r6) -> cubeP6/2
  CubeGrasp/9(pool_color) -> SplitRows_color/1(v)
  SplitRows_color/1(r1) -> cubeP1/3
  SplitRows_color/2(r2) -> cubeP2/3
  SplitRows_color/3(r3) -> cubeP3/3
  SplitRows_color/4(r4) -> cubeP4/3
  SplitRows_color/5(r5) -> cubeP5/3
  SplitRows_color/6(r6) -> cubeP6/3

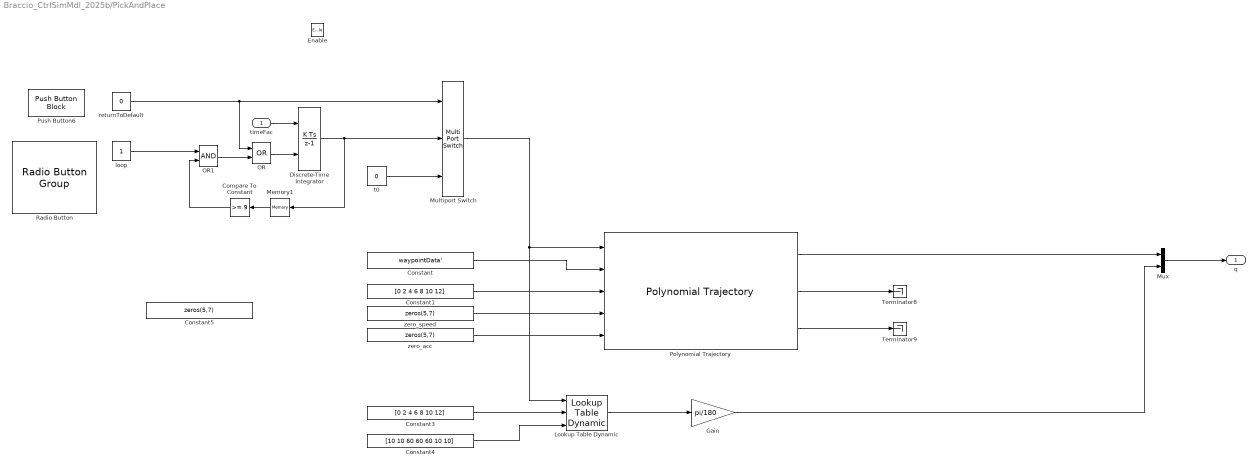
== system Braccio_CtrlSimMdl_2025b/PickAndPlace ==
  timeFac : Inport
  Enable : EnablePort
  Compare To Constant : simulink/Logic and Bit Operations/Compare To Constant  relop=>=  const=9  OutDataTypeStr=boolean
  Constant : Constant  Value=waypointData'  VectorParams1D=off
  Constant1 : Constant  Value=[0 2 4 6 8 10 12]
  Constant3 : Constant  Value=[0 2 4 6 8 10 12]
  Constant4 : Constant  Value=[10 10 60 60 60 10 10]
  Constant5 : Constant  Value=zeros(5,7)  VectorParams1D=off
  Discrete-Time Integrator : DiscreteIntegrator  ExternalReset=level  SampleTime=-1  ICPrevOutput=DiscIntNeverNeededParam  ICPrevScaledInput=DiscIntNeverNeededParam
  Gain : Gain  Gain=pi/180
  Lookup Table Dynamic : simulink/Lookup Tables/Lookup Table Dynamic  LookUpMeth=Interpolation-Use End Values  OutDataType=fixdt('double')  OutScaling=[]  OutputDataTypeScalingMode=Specify via dialog  OutDataTypeStr=double  DoSatur=off
  Memory1 : Memory  InheritSampleTime=on
  Multiport Switch : MultiPortSwitch  DataPortOrder=Zero-based contiguous  Inputs=2  zeroidx=on  SaturateOnIntegerOverflow=off  InputSameDT=off
  Mux : Mux  Inputs=2
  OR : Logic  Operator=OR  AllPortsSameDT=off  OutDataTypeStr=boolean
  OR1 : Logic  AllPortsSameDT=off  OutDataTypeStr=boolean
  Polynomial Trajectory : robotcorelib/Polynomial Trajectory  WaypointSource=External  Waypoints=[ 0, 2, 1, 5, 0; -1, 3, 1, 4, 4 ]  TimePoints=[ 0, 1, 2, 3, 4 ]  TimeInterval=[ 1, 4 ]  Method=Quintic Polynomial  ParameterSource=External  VelocityBoundaryCondition=zeros( 5, 6 )  AccelerationBoundaryCondition=zeros( 5, 6 )  SimulateUsing=Interpreted execution
  Push Button6 : PushButtonBlock  ButtonText=Default Pos  ButtonType=Latch  IconOnColor=[0.0, 0.39215686274509803, 0.0]  IconOffColor=[0.0, 1.0, 0.0]  OffValue=0.000000
  Radio Button : RadioButtonGroup  SelectedLabel=Loop ON  ButtonGroupName=Group
  Terminator8 : Terminator
  Terminator9 : Terminator
  loop : Constant  SampleTime=dt
  returnToDefault : Constant  Value=0  SampleTime=dt
  t0 : Constant  Value=0  SampleTime=dt
  zero_acc : Constant  Value=zeros(5,7)
  zero_speed : Constant  Value=zeros(5,7)
  q : Outport
  wires:
  Lookup Table Dynamic/1 -> Gain/1
  Mux/1 -> q/1
  Multiport Switch/1 -> Lookup Table Dynamic/1, Polynomial Trajectory/1
  OR1/1 -> OR/2
  Polynomial Trajectory/2 -> Terminator8/1
  loop/1 -> OR1/1
  zero_speed/1 -> Polynomial Trajectory/4
  returnToDefault/1 -> Multiport Switch/1, OR/1
  zero_acc/1 -> Polynomial Trajectory/5
  Memory1/1 -> Compare To Constant/1
  Constant1/1 -> Polynomial Trajectory/3
  Polynomial Trajectory/3 -> Terminator9/1
  OR/1 -> Discrete-Time Integrator/2
  Compare To Constant/1 -> OR1/2
  timeFac/1 -> Discrete-Time Integrator/1
  Polynomial Trajectory/1 -> Mux/1
  Discrete-Time Integrator/1 -> Multiport Switch/2, Memory1/1
  t0/1 -> Multiport Switch/3
  Constant3/1 -> Lookup Table Dynamic/2
  Constant4/1 -> Lookup Table Dynamic/3
  Gain/1 -> Mux/2
  Constant/1 -> Polynomial Trajectory/2

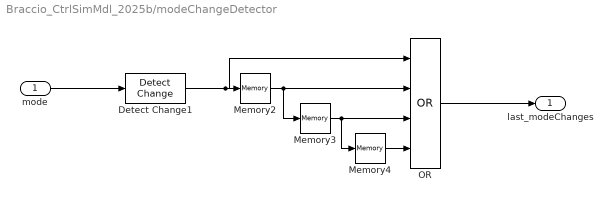
== system Braccio_CtrlSimMdl_2025b/modeChangeDetector ==
  mode : Inport
  Detect Change1 : simulink/Logic and Bit Operations/Detect Change  vinit=0  OutDataTypeStr=boolean
  Memory2 : Memory
  Memory3 : Memory
  Memory4 : Memory
  OR : Logic  Operator=OR  Inputs=4  AllPortsSameDT=off  OutDataTypeStr=boolean
  last_modeChanges : Outport
  wires:
  OR/1 -> last_modeChanges/1
  Memory2/1 -> Memory3/1, OR/2
  Memory3/1 -> Memory4/1, OR/3
  Memory4/1 -> OR/4
  Detect Change1/1 -> OR/1, Memory2/1
  mode/1 -> Detect Change1/1

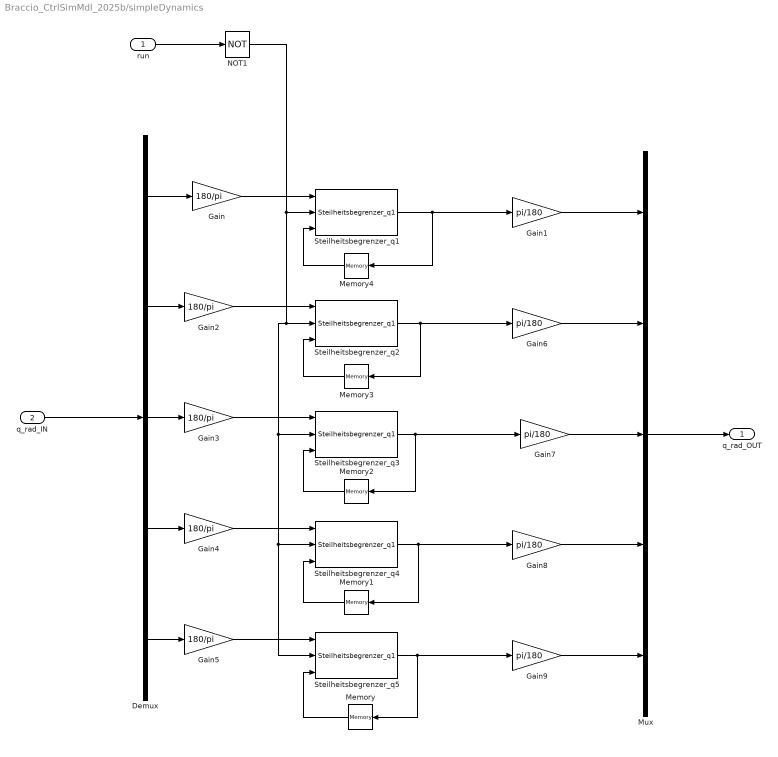
== system Braccio_CtrlSimMdl_2025b/simpleDynamics ==
  run : Inport
  q_rad_IN : Inport  Port=2
  Demux : Demux  Outputs=5
  Gain{,2..5} (5 alike) : Gain  Gain=180/pi
  Gain{1,6..9} (5 alike) : Gain  Gain=pi/180
  Memory : Memory
  Memory1 : Memory  InitialCondition=90
  Memory2 : Memory
  Memory3 : Memory  InitialCondition=90
  Memory4 : Memory
  Mux : Mux  Inputs=5
  NOT1 : Logic  Operator=NOT  IconShape=distinctive  AllPortsSameDT=off  OutDataTypeStr=boolean
  Steilheitsbegrenzer_q{1..5} (5 alike) : Braccio_lib/Steilheitsbegrenzer_q1  SystemSampleTime=-1  VariantActivationTime=update diagram  EmptyChoice=off  PassThrough=off  PassThroughVariantControl=(default)  EmptyChoiceVariantControl=(default)  AllowFlexibleInterface=on  Latency=0  AutoFrameSizeCalculation=off
  q_rad_OUT : Outport
  wires:
  Mux/1 -> q_rad_OUT/1
  Demux/2 -> Gain2/1
  Demux/1 -> Gain/1
  Demux/3 -> Gain3/1
  Demux/4 -> Gain4/1
  Demux/5 -> Gain5/1
  Gain1/1 -> Mux/1
  Gain6/1 -> Mux/2
  Gain7/1 -> Mux/3
  Gain8/1 -> Mux/4
  Gain9/1 -> Mux/5
  Gain/1 -> Steilheitsbegrenzer_q1/1
  Gain2/1 -> Steilheitsbegrenzer_q2/1
  Gain3/1 -> Steilheitsbegrenzer_q3/1
  Gain4/1 -> Steilheitsbegrenzer_q4/1
  Gain5/1 -> Steilheitsbegrenzer_q5/1
  Steilheitsbegrenzer_q1/1 -> Memory4/1, Gain1/1
  Steilheitsbegrenzer_q3/1 -> Gain7/1, Memory2/1
  Steilheitsbegrenzer_q5/1 -> Gain9/1, Memory/1
  q_rad_IN/1 -> Demux/1
  run/1 -> NOT1/1
  NOT1/1 -> Steilheitsbegrenzer_q1/2, Steilheitsbegrenzer_q3/2, Steilheitsbegrenzer_q5/2, Steilheitsbegrenzer_q4/2, Steilheitsbegrenzer_q2/2
  Steilheitsbegrenzer_q2/1 -> Memory3/1, Gain6/1
  Steilheitsbegrenzer_q4/1 -> Gain8/1, Memory1/1
  Memory/1 -> Steilheitsbegrenzer_q5/3
  Memory1/1 -> Steilheitsbegrenzer_q4/3
  Memory2/1 -> Steilheitsbegrenzer_q3/3
  Memory3/1 -> Steilheitsbegrenzer_q2/3
  Memory4/1 -> Steilheitsbegrenzer_q1/3

== matlab function Braccio_CtrlSimMdl_2025b/CubeInteraction/CubeGrasp ==
  data: T_tcp input; cube1_pos output; q_set input; mode input; respawn input; cube1_rot output; cube2_pos output; cube2_rot output; q6_vis output; graspIdx output; braccioCubes parameter; pool_pos output; pool_rot output; pool_color output; pool_transp output
function [cube1_pos, cube1_rot, cube2_pos, cube2_rot, q6_vis, graspIdx, pool_pos, pool_rot, pool_color, pool_transp] = CubeGrasp(T_tcp, q_set, mode, respawn, braccioCubes)
%CUBEGRASP Greifen/Absetzen/Respawning der Wuerfel, Reset bei Moduswechsel
%   T_tcp  4x4 TCP-Pose (Basis-KS), q_set 6x1 Sollwinkel inkl. q6 [rad]
%   respawn  1 = leere Startplaetze automatisch neu belegen
%   q6_vis 3x1 [q6; Wuerfelbreite; y-Mitte] fuer GripperVisu
%   Ausgaenge im Unreal-KS; pool_* zeilenweise aneinandergehaengt fuer cubeP1..cubePn
persistent modePrev
if isempty(modePrev)
    modePrev = mode;
end
reset = mode ~= modePrev;
modePrev = mode;
[p, r, col, tr, q6_vis, graspIdx] = Braccio_cubeGrasp(T_tcp, q_set(6), reset, respawn > 0, braccioCubes);
cube1_pos = p(1, :);
cube1_rot = r(1, :);
cube2_pos = p(2, :);
cube2_rot = r(2, :);
iPool = 3:size(p, 1);
pool_pos = reshape(p(iPool, :)', [], 1);
pool_rot = reshape(r(iPool, :)', [], 1);
pool_color = reshape(col(iPool, :)', [], 1);
pool_transp = tr(iPool);
